simulink model "statom_3_phase"  (R2025a)
settings: Solver=ode2  StartTime=0.0  StopTime=1  FixedStep=2e-6  RelTol=1e-3  EnableMultiTasking=on
undefined symbols (not defined in the file): Vsrc_LL
libraries: spsCurrentMeasurementLib x9, spsMosfetLib x6, spsVoltageMeasurementLib x5, spsSeriesRLCBranchLib x5, spsBreakerLib x3, simulink x1, spsIdealSwitchLib x1, spsThreePhaseSeriesRLCLoadLib x1, spsThreePhaseSourceLib x1, spspowerguiLib x1
settings Model: Creator=ankush  LastModifiedBy=SimuVerity Contributors
settings SolverCC: AlgebraicLoopSolver=TrustRegion
settings DataIOCC: LimitDataPoints=on  SaveFormat=Array  SignalLoggingSaveFormat=ModelDataLogs  ReturnWorkspaceOutputs=off
settings OptimizationCC: ExpressionDepthLimit=2147483647.0  LifeSpan=inf
settings DebuggingCC: UnderspecifiedInitializationDetection=Classic  MergeDetectMultiDrivingBlocksExec=none  SolverPrmCheckMsg=warning  FcnCallInpInsideContextMsg=warning  UnconnectedInputMsg=warning  UnconnectedOutputMsg=warning  UnconnectedLineMsg=warning  StateNameClashWarn=warning  SFUnexpectedBacktrackingDiag=warning  SFNoUnconditionalDefaultTransitionDiag=warning  SFExecutionAtInitializationDiag=none  ArithmeticOperatorsInVariantConditions=warning
settings HardwareCC: ProdBitPerPointer=32.0  ProdBitPerSizeT=32.0  ProdBitPerPtrDiffT=32.0  ProdLargestAtomicFloat=None  ProdIntDivRoundTo=Undefined  ProdEndianess=Unspecified  ProdWordSize=32.0  ProdHWDeviceType=32-bit Generic
settings ModelReferenceCC: PropagateSignalLabelsOutOfModel=off
settings SFSimCC: SimUseLocalCustomCode=off  CustomCodeUndefinedFunction=UseInterfaceOnly
settings RTWCC: RTWUseLocalCustomCode=off  GPUComputeCapability=3.5
settings CodeAppCC: StateflowObjectComments=on
settings GRTTargetCC: TargetLangStandard=C89/C90 (ANSI)  CombineOutputUpdateFcns=off  GRTInterface=on
settings ConfigComp: CovMetricSettings=dw  CovSaveCumulativeToWorkspaceVar=on  CovSaveSingleToWorkspaceVar=on  CovExternalEMLEnable=off

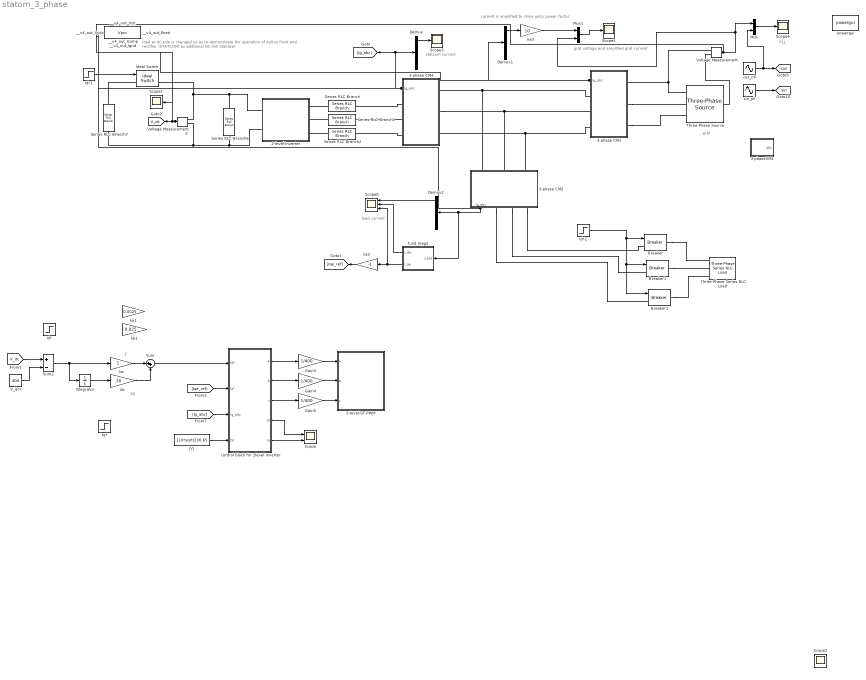
== system statom_3_phase ==
  note: 1
  note: 30
  note: grid
  note: statcom current
  note: grid voltage and amplified grid current
  note: load current
  note: PLL
  note: current is amplified to show unity power factor
  note: load at dc side is changed so as to demonstrate the operation of Active front
      |  end rectifier (STATCOM) as addtional DC-link Stablizer
  2-level-ST-PWM : Subsystem
  2-level-inverter : Subsystem
  3-phase CM1 : Subsystem
  3-phase CM2 : Subsystem
  3-phase CM4 : Subsystem
  3-phaseVM1 : Subsystem
  Breaker : spsBreakerLib/Breaker  InitialState=0  SwitchingTimes="[ 1/60  5/60 ]"  External=on  BreakerResistance=0.01  SnubberResistance=1e6  SnubberCapacitance=inf  Measurements=None  MoreParameters=off  NoBreakLoop=off
  Breaker1 : spsBreakerLib/Breaker  InitialState=0  SwitchingTimes="[ 1/60  5/60 ]"  External=on  BreakerResistance=0.01  SnubberResistance=1e6  SnubberCapacitance=inf  Measurements=None  MoreParameters=off  NoBreakLoop=off
  Breaker2 : spsBreakerLib/Breaker  InitialState=0  SwitchingTimes="[ 1/60  5/60 ]"  External=on  BreakerResistance=0.01  SnubberResistance=1e6  SnubberCapacitance=inf  Measurements=None  MoreParameters=off  NoBreakLoop=off
  Demux : Demux  Outputs=3
  Demux1 : Demux  Outputs=3
  Demux2 : Demux  Outputs=3
  Gain3 : Gain  Gain=1/400
  Gain4 : Gain  Gain=1/400
  Gain5 : Gain  Gain=1/400
  Id* : Step  Time=0.2  After=10  SampleTime=0
  Id*1 : Step  Time=0.7  SampleTime=0
  Id*2 : Step  Time=0.3  SampleTime=0
  Ideal Switch : spsIdealSwitchLib/Ideal Switch  Ron=0.001  Lon=0  IC=0  Rs=1e5  Cs=inf  Measurements=on
  Integrator : Integrator
  Iq* : Step  Time=0.7  After=0  SampleTime=0
  Mux : Mux  Inputs=2
  Mux1 : Mux  Inputs=2
  Scope : Scope  NumInputPorts=2
      settings: TimeSpan=1.4  ActiveDisplayYMinimum=0.6869  ActiveDisplayYMaximum=0.6882  DataLoggingVariableName=ScopeData3
  Scope{1,3..5} (4 alike) : Scope
      Scope1 settings: ActiveDisplayYMinimum=-6  ActiveDisplayYMaximum=7
      Scope3 settings: ActiveDisplayYMinimum=-6  ActiveDisplayYMaximum=7
      Scope4 settings: ActiveDisplayYMinimum=-6  ActiveDisplayYMaximum=7  DataLoggingVariableName=ScopeData4
      Scope5 settings: ActiveDisplayYMinimum=-6  ActiveDisplayYMaximum=7  DataLoggingVariableName=ScopeData5
  Scope2 : Scope  NumInputPorts=2
      settings: ActiveDisplayYMinimum=-5  ActiveDisplayYMaximum=5  DataLoggingVariableName=ScopeData2
  Scope6 : Scope  NumInputPorts=3
      settings: ActiveDisplayYMinimum=-6  ActiveDisplayYMaximum=7  DataLoggingVariableName=ScopeData6
  Series RLC Branch : spsSeriesRLCBranchLib/Series RLC Branch  LConnTagsString=__new0  RConnTagsString=__new0  BranchType=RL  Resistance=0.03  Inductance=3e-3  SetiL0=off  InitialCurrent=0  Capacitance=1e-6  Setx0=off  InitialVoltage=0  Measurements=None
  Series RLC Branch1 : spsSeriesRLCBranchLib/Series RLC Branch  LConnTagsString=__new0  RConnTagsString=__new0  BranchType=RL  Resistance=0.03  Inductance=3e-3  SetiL0=off  InitialCurrent=0  Capacitance=1e-6  Setx0=off  InitialVoltage=0  Measurements=None
  Series RLC Branch2 : spsSeriesRLCBranchLib/Series RLC Branch  LConnTagsString=__new0  RConnTagsString=__new0  BranchType=RL  Resistance=0.03  Inductance=3e-3  SetiL0=off  InitialCurrent=0  Capacitance=1e-6  Setx0=off  InitialVoltage=0  Measurements=None
  Series RLC Branch6 : spsSeriesRLCBranchLib/Series RLC Branch  LConnTagsString=__new0  RConnTagsString=__new0  BranchType=C  Resistance=0.03  Inductance=1e-3  SetiL0=off  InitialCurrent=0  Capacitance=2000e-6  Setx0=on  InitialVoltage=400  Measurements=None
  Series RLC Branch7 : spsSeriesRLCBranchLib/Series RLC Branch  LConnTagsString=__new0  RConnTagsString=__new0  BranchType=R  Resistance=100  Inductance=3e-3  SetiL0=off  InitialCurrent=0  Capacitance=1e-6  Setx0=off  InitialVoltage=0  Measurements=None
  Sum : Sum  Inputs=|++
  Sum2 : Sum  Inputs=+-
  Three-Phase Series RLC Load : spsThreePhaseSeriesRLCLoadLib/Three-Phase Series RLC Load  LConnTagsString=A|B|C  Configuration=Y (grounded)  NominalVoltage=110*sqrt(3)  Vabc=[1e3 1e3 1e3]  Vabcp=[1e3 1e3 1e3]  NominalFrequency=50  UnbalancedPower=off  ActivePower=P_load  InductivePower=Q_load  CapacitivePower=0  Pabc=[10e3 9e3 11e3]  QLabc=[100 90 110]  QCabc=[100 90 110]  Pabcp=[10e3 9e3 11e3]  QLabcp=[100 90 110]  QCabcp=[100 90 110]  Measurements=None  LoadType=constant Z
  Three-Phase Source : spsThreePhaseSourceLib/Three-Phase Source  InternalConnection=Yn  VoltagePhases=off  Voltage=Vsrc_LL  PhaseAngle=0  Voltage_phases=[25e3 25e3 25e3]/sqrt(3)  PhaseAngles_phases=[0 -120 +120]  Frequency=50  NonIdealSource=on  SpecifyImpedance=off  Resistance=0  Inductance=0  ShortCircuitLevel=100e6  BaseVoltage=25e3  XRratio=7  BusType=swing  Pref=10e3  Qref=0  Prefabc=[10e3, 10e3, 10e3]  Qrefabc=[0, 0, 0]  Qmin=-inf  Qmax=inf
  V_dc* : Constant  Value=400
  Voltage Measurement : spsVoltageMeasurementLib/Voltage Measurement  PhasorSimulation=off  OutputType=Complex  PSBequivalent=0
  Voltage Measurement2 : spsVoltageMeasurementLib/Voltage Measurement  PhasorSimulation=off  OutputType=Complex  PSBequivalent=0
  __v4_out_Icomp : ToWorkspace  VariableName=Icomp  SaveFormat=Timeseries  SampleTime=-1
  __v4_out_Igrid : ToWorkspace  VariableName=Igrid  SaveFormat=Timeseries  SampleTime=-1
  __v4_out_Iload : ToWorkspace  VariableName=Iload  SaveFormat=Timeseries  SampleTime=-1
  __v4_out_Vdc : ToWorkspace  VariableName=Vdc  SaveFormat=Timeseries  SampleTime=-1
  __v4_out_Vpcc : ToWorkspace  VariableName=Vpcc  SaveFormat=Timeseries  SampleTime=-1
  control block for 2level inverter : Subsystem
  cos_pll : Sin  Frequency=2*pi*50  Phase=pi/2  SampleTime=0
  fund mag2 : Subsystem
  ka : Gain
  ka1 : Gain  Gain=0.0025
  ka2 : Gain  Gain=-1
  ka3 : Gain  Gain=10
  kb : Gain  Gain=30
  kb1 : Gain  Gain=0.025
  powergui : spspowerguiLib/powergui  Priority=1  SimulationMode=Discrete  SampleTime=2e-6  frequency=60  Iterations=50  frequencyindice=50  Pbase=100e6  ErrMax=1e-4  UnitsV=kV  UnitsW=MW  buscounter=0  FunctionMessages=off  echomessages=off  EnableUseOfTLC=off  CurrentSourceSwitches=off  DisableSnubberDevices=off  DisableRonSwitches=off  DisableVfSwitches=off  DisplayEquations=off  AutomaticDiscreteSolvers=off  SolverType=Tustin/Backward Euler (TBE)  Interpol=off  ExternalGateDelay=off  methode=off  Ts=100  x0status=blocks  SPID=off  SwTol=0  HookPort=off  NonlinearTolerance=1e-4  nMaxIteration=100  ContinueOnMaxIteration=off  RestoreLinks=warning  ResistiveCurrentMeasurement=off  Frange=[0:2:500]  Ylog=off  Xlog=on  ShowGrid=off  save=off  variable=ZData  structure=ref_current  ZoomFFT=off  StartTime=0.0  cycles=50  DisplayStyle=1  fundamental=50  FreqAxis=off  MaxFrequency=1000  frequencyindicesteady=1  RmsSteady=1  display=off
  sin_pll : Sin  Frequency=2*pi*50  SampleTime=0
  |V| : Constant  Value=110*sqrt(2)/0.65
  tag scope: V_dc=global, cos=global, sin=global
  wires:
  sin_pll/1 -> [sin]
  cos_pll/1 -> [cos], Mux/2
  [Ig_abc] -> control block for 2level inverter/3(Ig_abc)
  Gain3/1 -> 2-level-ST-PWM/1(a)
  Gain4/1 -> 2-level-ST-PWM/2(b)
  Gain5/1 -> 2-level-ST-PWM/3(c)
  control block for 2level inverter/1(a) -> Gain3/1
  control block for 2level inverter/2(b) -> Gain4/1
  control block for 2level inverter/3(c) -> Gain5/1
  3-phase CM4/1(Ig_abc) -> [Ig_abc], Demux/1, __v4_out_Icomp/1
  Sum/1 -> control block for 2level inverter/1(Id*)
  Voltage Measurement2/1 -> [V_dc], Scope1/1, __v4_out_Vdc/1
  Integrator/1 -> kb/1
  Sum2/1 -> Integrator/1, ka/1
  ka/1 -> Sum/1
  kb/1 -> Sum/2
  [V_dc] -> Sum2/1
  V_dc*/1 -> Sum2/2
  Id*1/1 -> Ideal Switch/1
  |V|/1 -> control block for 2level inverter/4(|V|)
  Demux/1 -> Scope3/1
  control block for 2level inverter/4(Id) -> Scope/1
  control block for 2level inverter/5(Iq) -> Scope/2
  Voltage Measurement/1 -> Mux/1, Mux1/2, __v4_out_Vpcc/1
  Mux/1 -> Scope4/1
  3-phase CM1/1(Ig_abc) -> Demux1/1, __v4_out_Igrid/1
  Id*2/1 -> Breaker/1, Breaker1/1, Breaker2/1
  3-phase CM2/1(Ig_abc) -> Demux2/1, fund mag2/1(I_abc), __v4_out_Iload/1
  Demux2/1 -> Scope6/1
  fund mag2/1(I_de) -> Scope6/2
  fund mag2/2(I_qe) -> Scope6/3, ka2/1
  [Iqe_ref] -> control block for 2level inverter/2(Iq*)
  Demux1/1 -> ka3/1
  Mux1/1 -> Scope5/1
  ka2/1 -> [Iqe_ref]
  ka3/1 -> Mux1/1
  connections:
  Series RLC Branch/LConn1 -- 2-level-inverter/LConn1
  Series RLC Branch1/LConn1 -- 2-level-inverter/LConn2
  Series RLC Branch2/LConn1 -- 2-level-inverter/LConn3
  3-phase CM4/RConn3 -- Series RLC Branch2/RConn1
  3-phase CM4/RConn2 -- Series RLC Branch1/RConn1
  3-phase CM4/RConn1 -- Series RLC Branch/RConn1
  Voltage Measurement/LConn1 -- Three-Phase Source/RConn1 -- 3-phase CM1/LConn1
  Ideal Switch/RConn1 -- Series RLC Branch6/LConn1 -- 2-level-inverter/RConn1 -- Voltage Measurement2/LConn1
  2-level-inverter/RConn2 -- Series RLC Branch6/RConn1 -- Series RLC Branch7/RConn1 -- Voltage Measurement2/LConn2
  Series RLC Branch7/LConn1 -- Ideal Switch/LConn1
  Three-Phase Source/LConn1 -- Voltage Measurement/LConn2
  3-phase CM1/LConn2 -- Three-Phase Source/RConn2
  3-phase CM1/LConn3 -- Three-Phase Source/RConn3
  3-phase CM1/RConn1 -- 3-phase CM4/LConn1 -- 3-phase CM2/LConn1
  3-phase CM4/LConn2 -- 3-phase CM1/RConn2 -- 3-phase CM2/LConn2
  3-phase CM1/RConn3 -- 3-phase CM4/LConn3 -- 3-phase CM2/LConn3
  3-phase CM2/RConn3 -- Breaker/LConn1
  3-phase CM2/RConn2 -- Breaker1/LConn1
  3-phase CM2/RConn1 -- Breaker2/LConn1
  Breaker1/RConn1 -- Three-Phase Series RLC Load/LConn2
  Breaker/RConn1 -- Three-Phase Series RLC Load/LConn1
  Breaker2/RConn1 -- Three-Phase Series RLC Load/LConn3

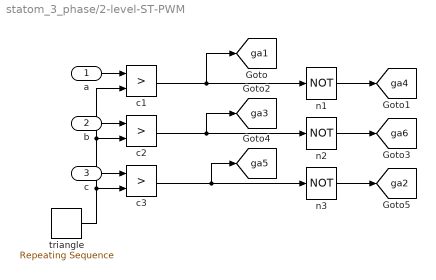
== system statom_3_phase/2-level-ST-PWM ==
  a : Inport
  b : Inport  Port=2
  c : Inport  Port=3
  c1 : RelationalOperator  Operator=>  OutDataTypeStr=boolean  InputSameDT=off
  c2 : RelationalOperator  Operator=>  OutDataTypeStr=boolean  InputSameDT=off
  c3 : RelationalOperator  Operator=>  OutDataTypeStr=boolean  InputSameDT=off
  n1 : Logic  Operator=NOT  AllPortsSameDT=off  OutDataTypeStr=boolean
  n2 : Logic  Operator=NOT  AllPortsSameDT=off  OutDataTypeStr=boolean
  n3 : Logic  Operator=NOT  AllPortsSameDT=off  OutDataTypeStr=boolean
  triangle : simulink/Sources/Repeating Sequence  rep_seq_t=[0 0.5e-4 1e-4]  rep_seq_y=[1 -1 1]
  tag scope: ga1=global, ga2=global, ga3=global, ga4=global, ga5=global, ga6=global
  wires:
  triangle/1 -> c3/2, c2/2, c1/2
  c1/1 -> n1/1, [ga1]
  c2/1 -> n2/1, [ga3]
  c3/1 -> n3/1, [ga5]
  n1/1 -> [ga4]
  n2/1 -> [ga6]
  n3/1 -> [ga2]
  a/1 -> c1/1
  b/1 -> c2/1
  c/1 -> c3/1

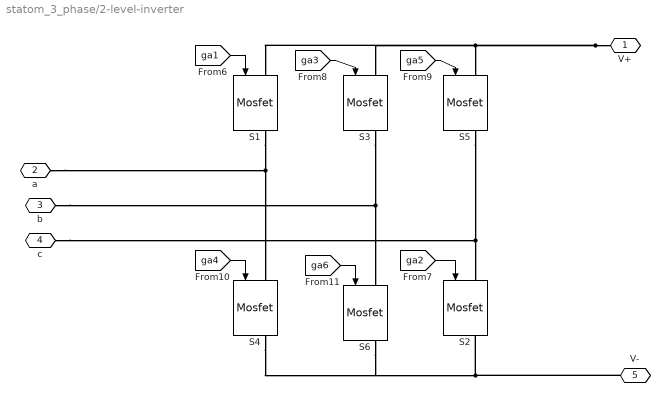
== system statom_3_phase/2-level-inverter ==
  S{1..6} (6 alike) : spsMosfetLib/Mosfet  Ron=0.1  Lon=0  Rd=0.01  Vfd=0  IC=0  Rs=1e5  Cs=inf  Measurements=on
  V+ : PMIOPort  Side=Right
  a : PMIOPort  Port=2  Side=Left
  b : PMIOPort  Port=3  Side=Left
  c : PMIOPort  Port=4  Side=Left
  V- : PMIOPort  Port=5  Side=Right
  wires:
  [ga6] -> S6/1
  [ga4] -> S4/1
  [ga5] -> S5/1
  [ga3] -> S3/1
  [ga2] -> S2/1
  [ga1] -> S1/1
  connections:
  b/RConn1 -- S6/LConn1 -- S3/RConn1
  V-/RConn1 -- S2/RConn1 -- S6/RConn1 -- S4/RConn1
  c/RConn1 -- S5/RConn1 -- S2/LConn1
  a/RConn1 -- S4/LConn1 -- S1/RConn1
  V+/RConn1 -- S3/LConn1 -- S1/LConn1 -- S5/LConn1

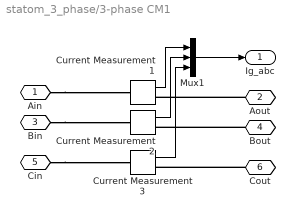
== system statom_3_phase/3-phase CM1 ==
  Current Measurement1 : spsCurrentMeasurementLib/Current Measurement  PhasorSimulation=off  OutputType=Complex  PSBequivalent=0
  Current Measurement2 : spsCurrentMeasurementLib/Current Measurement  PhasorSimulation=off  OutputType=Complex  PSBequivalent=0
  Current Measurement3 : spsCurrentMeasurementLib/Current Measurement  PhasorSimulation=off  OutputType=Complex  PSBequivalent=0
  Mux1 : Mux  Inputs=3
  Ain : PMIOPort  Side=Right
  Aout : PMIOPort  Port=2  Side=Left
  Bin : PMIOPort  Port=3  Side=Right
  Bout : PMIOPort  Port=4  Side=Left
  Cin : PMIOPort  Port=5  Side=Right
  Cout : PMIOPort  Port=6  Side=Left
  Ig_abc : Outport
  wires:
  Mux1/1 -> Ig_abc/1
  Current Measurement3/1 -> Mux1/3
  Current Measurement2/1 -> Mux1/2
  Current Measurement1/1 -> Mux1/1
  connections:
  Cout/RConn1 -- Current Measurement3/RConn1
  Cin/RConn1 -- Current Measurement3/LConn1
  Bout/RConn1 -- Current Measurement2/RConn1
  Bin/RConn1 -- Current Measurement2/LConn1
  Aout/RConn1 -- Current Measurement1/RConn1
  Ain/RConn1 -- Current Measurement1/LConn1

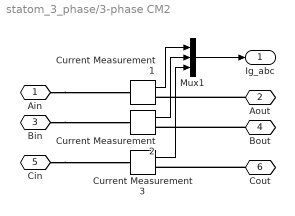
== system statom_3_phase/3-phase CM2 ==
  Current Measurement1 : spsCurrentMeasurementLib/Current Measurement  PhasorSimulation=off  OutputType=Complex  PSBequivalent=0
  Current Measurement2 : spsCurrentMeasurementLib/Current Measurement  PhasorSimulation=off  OutputType=Complex  PSBequivalent=0
  Current Measurement3 : spsCurrentMeasurementLib/Current Measurement  PhasorSimulation=off  OutputType=Complex  PSBequivalent=0
  Mux1 : Mux  Inputs=3
  Ain : PMIOPort  Side=Right
  Aout : PMIOPort  Port=2  Side=Left
  Bin : PMIOPort  Port=3  Side=Right
  Bout : PMIOPort  Port=4  Side=Left
  Cin : PMIOPort  Port=5  Side=Right
  Cout : PMIOPort  Port=6  Side=Left
  Ig_abc : Outport
  wires:
  Current Measurement1/1 -> Mux1/1
  Current Measurement2/1 -> Mux1/2
  Current Measurement3/1 -> Mux1/3
  Mux1/1 -> Ig_abc/1
  connections:
  Ain/RConn1 -- Current Measurement1/LConn1
  Aout/RConn1 -- Current Measurement1/RConn1
  Bin/RConn1 -- Current Measurement2/LConn1
  Bout/RConn1 -- Current Measurement2/RConn1
  Cin/RConn1 -- Current Measurement3/LConn1
  Cout/RConn1 -- Current Measurement3/RConn1

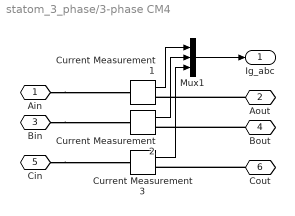
== system statom_3_phase/3-phase CM4 ==
  Current Measurement1 : spsCurrentMeasurementLib/Current Measurement  PhasorSimulation=off  OutputType=Complex  PSBequivalent=0
  Current Measurement2 : spsCurrentMeasurementLib/Current Measurement  PhasorSimulation=off  OutputType=Complex  PSBequivalent=0
  Current Measurement3 : spsCurrentMeasurementLib/Current Measurement  PhasorSimulation=off  OutputType=Complex  PSBequivalent=0
  Mux1 : Mux  Inputs=3
  Ain : PMIOPort  Side=Right
  Aout : PMIOPort  Port=2  Side=Left
  Bin : PMIOPort  Port=3  Side=Right
  Bout : PMIOPort  Port=4  Side=Left
  Cin : PMIOPort  Port=5  Side=Right
  Cout : PMIOPort  Port=6  Side=Left
  Ig_abc : Outport
  wires:
  Current Measurement1/1 -> Mux1/1
  Current Measurement2/1 -> Mux1/2
  Current Measurement3/1 -> Mux1/3
  Mux1/1 -> Ig_abc/1
  connections:
  Ain/RConn1 -- Current Measurement1/LConn1
  Aout/RConn1 -- Current Measurement1/RConn1
  Bin/RConn1 -- Current Measurement2/LConn1
  Bout/RConn1 -- Current Measurement2/RConn1
  Cin/RConn1 -- Current Measurement3/LConn1
  Cout/RConn1 -- Current Measurement3/RConn1

== system statom_3_phase/3-phaseVM1 ==
  Mux : Mux  Inputs=3
  Voltage Measurement : spsVoltageMeasurementLib/Voltage Measurement  PhasorSimulation=off  OutputType=Complex  PSBequivalent=0
  Voltage Measurement1 : spsVoltageMeasurementLib/Voltage Measurement  PhasorSimulation=off  OutputType=Complex  PSBequivalent=0
  Voltage Measurement2 : spsVoltageMeasurementLib/Voltage Measurement  PhasorSimulation=off  OutputType=Complex  PSBequivalent=0
  n : PMIOPort  Side=Left
  a : PMIOPort  Port=2  Side=Left
  b : PMIOPort  Port=3  Side=Left
  c : PMIOPort  Port=4  Side=Left
  abc : Outport
  wires:
  Voltage Measurement1/1 -> Mux/2
  Voltage Measurement2/1 -> Mux/3
  Mux/1 -> abc/1
  Voltage Measurement/1 -> Mux/1
  connections:
  c/RConn1 -- Voltage Measurement2/LConn1
  b/RConn1 -- Voltage Measurement1/LConn1
  a/RConn1 -- Voltage Measurement/LConn1
  Voltage Measurement2/LConn2 -- Voltage Measurement1/LConn2 -- Voltage Measurement/LConn2 -- n/RConn1

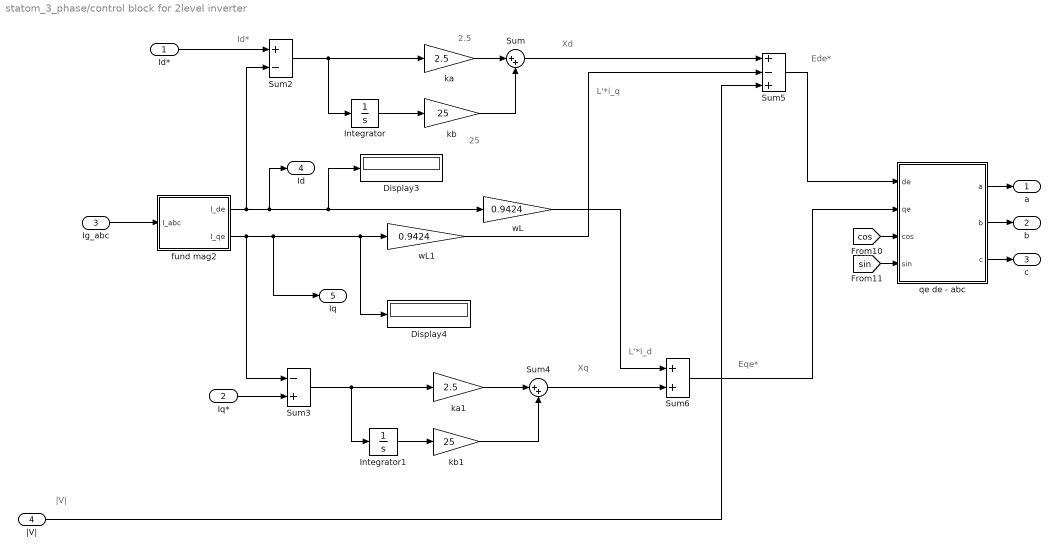
== system statom_3_phase/control block for 2level inverter ==
  note: |V|
  note: Id*
  note: Xd
  note: Xq
  note: L'*i_q
  note: L'*i_d
  note: Ede*
  note: Eqe*
  note: 2.5
  note: 25
  Id* : Inport
  Iq* : Inport  Port=2
  Ig_abc : Inport  Port=3
  |V| : Inport  Port=4
  Display3 : Display
  Display4 : Display
  Integrator : Integrator
  Integrator1 : Integrator
  Sum : Sum  Inputs=|++
  Sum2 : Sum  Inputs=+-
  Sum3 : Sum  Inputs=-+
  Sum4 : Sum  Inputs=|++
  Sum5 : Sum  Inputs=+-+
  Sum6 : Sum
  fund mag2 : Subsystem
  ka : Gain  Gain=2.5
  ka1 : Gain  Gain=2.5
  kb : Gain  Gain=25
  kb1 : Gain  Gain=25
  qe de - abc : Subsystem
  wL : Gain  Gain=0.9424
  wL1 : Gain  Gain=0.9424
  a : Outport
  b : Outport  Port=2
  c : Outport  Port=3
  Id : Outport  Port=4
  Iq : Outport  Port=5
  wires:
  |V|/1 -> Sum5/3
  fund mag2/1(I_de) -> Sum2/2, Display3/1, wL/1, Id/1
  fund mag2/2(I_qe) -> Sum3/1, Display4/1, wL1/1, Iq/1
  Integrator/1 -> kb/1
  Sum2/1 -> Integrator/1, ka/1
  ka/1 -> Sum/1
  kb/1 -> Sum/2
  Sum/1 -> Sum5/1
  Integrator1/1 -> kb1/1
  Sum3/1 -> Integrator1/1, ka1/1
  ka1/1 -> Sum4/1
  kb1/1 -> Sum4/2
  Sum4/1 -> Sum6/2
  wL1/1 -> Sum5/2
  wL/1 -> Sum6/1
  Iq*/1 -> Sum3/2
  Ig_abc/1 -> fund mag2/1(I_abc)
  Id*/1 -> Sum2/1
  [cos] -> qe de - abc/3(cos)
  [sin] -> qe de - abc/4(sin)
  Sum6/1 -> qe de - abc/2(qe)
  Sum5/1 -> qe de - abc/1(de)
  qe de - abc/1(a) -> a/1
  qe de - abc/2(b) -> b/1
  qe de - abc/3(c) -> c/1

== system statom_3_phase/fund mag2 ==
  I_abc : Inport
  Transfer Fcn : TransferFcn  Denominator=[0.01 1]
  Transfer Fcn1 : TransferFcn  Denominator=[0.01 1]
  abc - qd1 : Subsystem
  qd - qe de1 : Subsystem
  I_de : Outport
  I_qe : Outport  Port=2
  wires:
  abc - qd1/1(d) -> qd - qe de1/1(d)
  abc - qd1/2(q) -> qd - qe de1/2(q)
  [cos] -> qd - qe de1/3(cos)
  [sin] -> qd - qe de1/4(sin)
  I_abc/1 -> abc - qd1/1(abc)
  qd - qe de1/2(de) -> Transfer Fcn1/1
  qd - qe de1/1(qe) -> Transfer Fcn/1
  Transfer Fcn/1 -> I_de/1
  Transfer Fcn1/1 -> I_qe/1

== system statom_3_phase/control block for 2level inverter/fund mag2 ==
  I_abc : Inport
  Transfer Fcn : TransferFcn  Denominator=[0.01 1]
  Transfer Fcn1 : TransferFcn  Denominator=[0.01 1]
  abc - qd1 : Subsystem
  qd - qe de1 : Subsystem
  I_de : Outport
  I_qe : Outport  Port=2
  wires:
  abc - qd1/1(d) -> qd - qe de1/1(d)
  abc - qd1/2(q) -> qd - qe de1/2(q)
  [cos] -> qd - qe de1/3(cos)
  [sin] -> qd - qe de1/4(sin)
  I_abc/1 -> abc - qd1/1(abc)
  qd - qe de1/2(de) -> Transfer Fcn1/1
  qd - qe de1/1(qe) -> Transfer Fcn/1
  Transfer Fcn/1 -> I_de/1
  Transfer Fcn1/1 -> I_qe/1

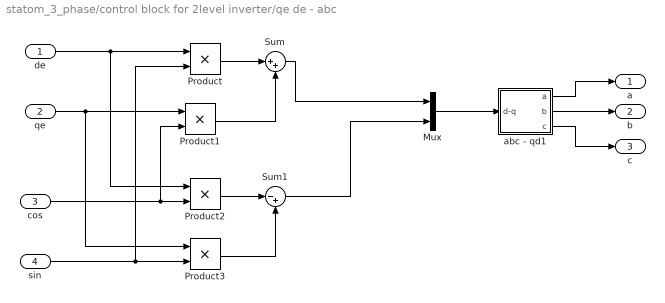
== system statom_3_phase/control block for 2level inverter/qe de - abc ==
  de : Inport
  qe : Inport  Port=2
  cos : Inport  Port=3
  sin : Inport  Port=4
  Mux : Mux  Inputs=2
  Product{,1..3} (4 alike) : Product  RndMeth=Zero
  Sum : Sum  Inputs=|++
  Sum1 : Sum  Inputs=|-+
  abc - qd1 : Subsystem
  a : Outport
  b : Outport  Port=2
  c : Outport  Port=3
  wires:
  Product/1 -> Sum/1
  Product1/1 -> Sum/2
  Product2/1 -> Sum1/1
  Product3/1 -> Sum1/2
  de/1 -> Product/1, Product2/1
  Sum/1 -> Mux/1
  sin/1 -> Product/2, Product3/2
  cos/1 -> Product1/2, Product2/2
  qe/1 -> Product1/1, Product3/1
  Sum1/1 -> Mux/2
  Mux/1 -> abc - qd1/1(d-q)
  abc - qd1/2(b) -> b/1
  abc - qd1/3(c) -> c/1
  abc - qd1/1(a) -> a/1

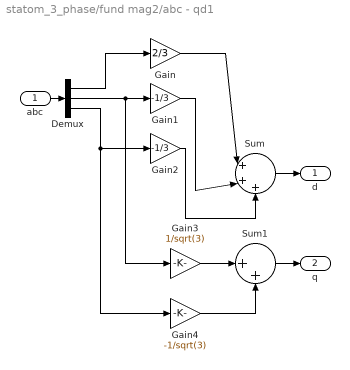
== system statom_3_phase/fund mag2/abc - qd1 ==
  abc : Inport
  Demux : Demux  Outputs=3
  Gain : Gain  Gain=2/3
  Gain1 : Gain  Gain=-1/3
  Gain2 : Gain  Gain=-1/3
  Gain3 : Gain  Gain=1/sqrt(3)
  Gain4 : Gain  Gain=-1/sqrt(3)
  Sum : Sum  Inputs=|+++
  Sum1 : Sum  Inputs=|++
  d : Outport
  q : Outport  Port=2
  wires:
  Demux/3 -> Gain4/1, Gain2/1
  Demux/2 -> Gain3/1, Gain1/1
  Sum1/1 -> q/1
  Sum/1 -> d/1
  Gain3/1 -> Sum1/1
  Gain4/1 -> Sum1/2
  Gain2/1 -> Sum/3
  Gain1/1 -> Sum/2
  Gain/1 -> Sum/1
  Demux/1 -> Gain/1
  abc/1 -> Demux/1

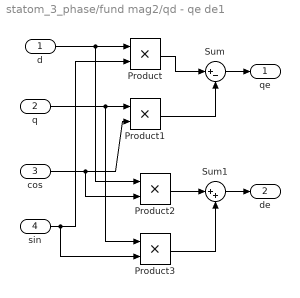
== system statom_3_phase/fund mag2/qd - qe de1 ==
  d : Inport
  q : Inport  Port=2
  cos : Inport  Port=3
  sin : Inport  Port=4
  Product{,1..3} (4 alike) : Product  RndMeth=Zero
  Sum : Sum  Inputs=|+-
  Sum1 : Sum  Inputs=|++
  qe : Outport
  de : Outport  Port=2
  wires:
  sin/1 -> Product3/2, Product/2
  cos/1 -> Product2/2, Product1/2
  Product/1 -> Sum/1
  Product1/1 -> Sum/2
  Product2/1 -> Sum1/1
  Product3/1 -> Sum1/2
  d/1 -> Product/1, Product2/1
  q/1 -> Product1/1, Product3/1
  Sum/1 -> qe/1
  Sum1/1 -> de/1

== system statom_3_phase/control block for 2level inverter/fund mag2/abc - qd1 ==
  abc : Inport
  Demux : Demux  Outputs=3
  Gain : Gain  Gain=2/3
  Gain1 : Gain  Gain=-1/3
  Gain2 : Gain  Gain=-1/3
  Gain3 : Gain  Gain=1/sqrt(3)
  Gain4 : Gain  Gain=-1/sqrt(3)
  Sum : Sum  Inputs=|+++
  Sum1 : Sum  Inputs=|++
  d : Outport
  q : Outport  Port=2
  wires:
  Demux/3 -> Gain4/1, Gain2/1
  Demux/2 -> Gain3/1, Gain1/1
  Sum1/1 -> q/1
  Sum/1 -> d/1
  Gain3/1 -> Sum1/1
  Gain4/1 -> Sum1/2
  Gain2/1 -> Sum/3
  Gain1/1 -> Sum/2
  Gain/1 -> Sum/1
  Demux/1 -> Gain/1
  abc/1 -> Demux/1

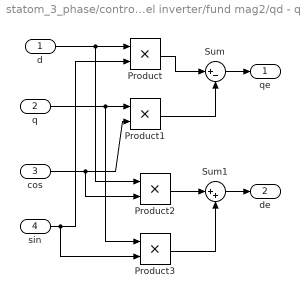
== system statom_3_phase/control block for 2level inverter/fund mag2/qd - qe de1 ==
  d : Inport
  q : Inport  Port=2
  cos : Inport  Port=3
  sin : Inport  Port=4
  Product{,1..3} (4 alike) : Product  RndMeth=Zero
  Sum : Sum  Inputs=|+-
  Sum1 : Sum  Inputs=|++
  qe : Outport
  de : Outport  Port=2
  wires:
  sin/1 -> Product3/2, Product/2
  cos/1 -> Product2/2, Product1/2
  Product/1 -> Sum/1
  Product1/1 -> Sum/2
  Product2/1 -> Sum1/1
  Product3/1 -> Sum1/2
  d/1 -> Product/1, Product2/1
  q/1 -> Product1/1, Product3/1
  Sum/1 -> qe/1
  Sum1/1 -> de/1

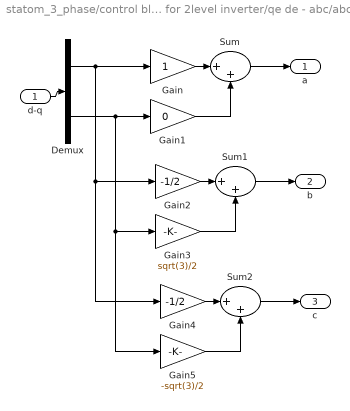
== system statom_3_phase/control block for 2level inverter/qe de - abc/abc - qd1 ==
  d-q : Inport
  Demux : Demux  Outputs=2
  Gain : Gain
  Gain1 : Gain  Gain=0
  Gain2 : Gain  Gain=-1/2
  Gain3 : Gain  Gain=sqrt(3)/2
  Gain4 : Gain  Gain=-1/2
  Gain5 : Gain  Gain=-sqrt(3)/2
  Sum : Sum  Inputs=|++
  Sum1 : Sum  Inputs=|++
  Sum2 : Sum  Inputs=|++
  a : Outport
  b : Outport  Port=2
  c : Outport  Port=3
  wires:
  d-q/1 -> Demux/1
  Demux/1 -> Gain/1, Gain2/1, Gain4/1
  Gain/1 -> Sum/1
  Demux/2 -> Gain1/1, Gain3/1, Gain5/1
  Gain1/1 -> Sum/2
  Sum/1 -> a/1
  Gain2/1 -> Sum1/1
  Gain3/1 -> Sum1/2
  Sum1/1 -> b/1
  Gain4/1 -> Sum2/1
  Gain5/1 -> Sum2/2
  Sum2/1 -> c/1
